simulink library "AFCToolbox"  (R2025b)
settings: Solver=VariableStepAuto  StartTime=0.0  StopTime=10.0  RelTol=1e-3
undefined symbols (not defined in the file or in its folder): AFC5Toolbox_SimuMoudle, ax, ay, az, C_d, C_dm, C_m, C_t, Control, d, declination_table, dp0, dp1, dp2, dp3, dt, euler_0, g0, I_xyz, inclination_table, J_m, lmd_high, lmd_low, lp_acc_knoise, lp_acc_max, lp_acc_min, lp_acc_seed, lp_GPS_BL_max, lp_GPS_BL_min, lp_GPS_H_max, lp_GPS_H_min, lp_GPS_knoise, lp_GPS_seed, lp_GPS_vel_max, lp_GPS_vel_min, lp_gyro_knoise, lp_gyro_max, lp_gyro_min, lp_gyro_seed, lp_hf_vwind, lp_hs_vwind_interp, lp_kaerorho, lp_kaeroT, lp_kIxyz, lp_kmass, lp_momentx_A0, lp_momentx_Af, lp_momentx_ts, lp_momenty_A0, lp_momenty_Af, lp_momenty_ts, lp_momentz_A0, lp_momentz_Af, lp_momentz_ts, lp_vf_vwind, lp_vs_vwind_interp, lp_vwind_thetax, lp_vwind_thetaz, mass, MB_states ... (+52)
libraries: $bdroot x104, simulink x75, etargetslib x32, sharedtransform x13, simulink_extras x12, dspstat3 x11, aerolibconvert2 x9, aerolibtransform2 x3, aerolibutil x2, matrix_library x1
(part 2 of 11)

== system AFCToolbox/SimuMoudle ==
  Equations of Motion1 : Subsystem  AncestorBlock=AFC5Toolbox_SimuMoudle/SimuMoudle/Equations of Motion1  mask(Equations of Motion){}
      mask init:
      | % port_label('input', 1, 'P+R+mg+F_c','texmode','on')
      | % port_label('input', 2, 'M_s_t+M_d+M_c+M\prime_r_e_l+M\prime_k','texmode','on')
      | % port_label('output', 1, 'V_G','texmode','on')
      | % port_label('output', 2, 'P_G','texmode','on')
      | % port_label('output', 3, 'R_0 _G','texmode','on')
      | % port_label('output', 4, 'G_B','texmode','on')
      | % port_label('output', 5, '\omega_T_1','texmode','on')
      | % port_label('output', 6, '\phi\prime \psi\prime \gamma\prime','texmode','on')
      | % port_label('output', 7, '\phi \psi \gamma','texmode','on')
      mask DialogControl Container1 Prompt: Equations of Motion
  Forces & Moments1 : Subsystem  AncestorBlock=AFC5Toolbox_SimuMoudle/SimuMoudle/Forces & Moments1
      mask DialogControl DescGroupVar Prompt: Forces & Moments
  LLA2XYZ : Subsystem  AncestorBlock=AFC5Toolbox_SimuMoudle/SimuMoudle/LLA2XYZ
      mask DialogControl DescGroupVar Prompt: LLA2BLH
      mask DialogControl DescTextVar Prompt: 将东北天坐标系的GPS_LLA转换为Pos_xyz
  Position-Control : Subsystem  AncestorBlock=AFC5Toolbox_SimuMoudle/SimuMoudle/Position-Control
      mask DialogControl DescGroupVar Prompt: 航线控制
      mask DialogControl DescTextVar Prompt: P0: 预设的无人机位置控制指令
  SimuBaro : Subsystem  AncestorBlock=AFC5Toolbox_SimuMoudle/SimuMoudle/SimuBaro  mask{lp_GPS_sample_time=0.01}
      mask prompts: lp_GPS_sample_time "采样时间："
      mask DialogControl DescGroupVar Prompt: 气压计模拟模块
      mask DialogControl DescTextVar Prompt: 本模块能够模拟仿真如下气压计信息：Time -- 模块时间（ms）;Press -- 气压（Pa）;H -- 高度（m）;Temp -- 温度（°）；
      mask DialogControl DescTextVar_copy Prompt: 所用时钟使用仿真时间代替；其中以下无法仿真使用常数暂代：Temp = 1;
  SimuComIn_ByteUnpack : Subsystem  AncestorBlock=AFC5Toolbox_SimuMoudle/SimuMoudle/SimuComIn_ByteUnpack  mask{para_count=4}
      mask prompts: para_count "数据位数："
      mask DialogControl DescGroupVar Prompt: SimuComIn_ByteUnpack
      mask DialogControl DescTextVar Prompt: 接收SimuCom应用层协议的数据，并分离出数据位。
  SimuComOut_BytePack : Subsystem  AncestorBlock=AFC5Toolbox_SimuMoudle/SimuMoudle/SimuComOut_BytePack
      mask DialogControl DescGroupVar Prompt: SimuComOut_BytePack
      mask DialogControl DescTextVar Prompt: 该模块将para数据位打包，适应SimuCom应用层协议。
      mask DialogControl DescTextVar_copy Prompt: para: 发送数据
  SimuGps : Subsystem  AncestorBlock=AFC5Toolbox_SimuMoudle/SimuMoudle/SimuGps  mask{lp_GPS_sample_time=0.01}
      mask prompts: lp_GPS_sample_time "采样时间："
      mask DialogControl DescGroupVar Prompt: GPS模拟模块
      mask DialogControl DescTextVar Prompt: 本模块能够模拟仿真如下GPS信息：Lat -- 维度，北纬为正（单位：°）；Lon -- 经度，东经为正（单位：°）;Alt -- 海拔高度（单位：m）;Vx -- 表示正北速度；Vy -- 表示正东速度；Vz -- 表示向上速度；Vgnd -- 地速；HeadAng -- 真北航向角（单位：°）；STS -- GPS状态；stasN -- 卫星个数；hdop -- 水平精度因子。
      mask DialogControl DescTextVar_copy Prompt: 所有时钟使用仿真时间代替；其中以下无法仿真使用常数暂代：Sts = 1;StasN = 2;hdop = 3;
  SimuICM : Subsystem  AncestorBlock=AFC5Toolbox_SimuMoudle/SimuMoudle/SimuICM  mask{lp_sample_time=0.01}
      mask prompts: lp_sample_time "采样时间："
      mask DialogControl DescGroupVar Prompt: 惯性测量模拟模块
      mask DialogControl DescTextVar Prompt: 本模块能够模拟仿真陀螺仪和加速度计如下信息：Tim -- 模拟时间（ms）；Wx Wy Wz -- 角速率（°/s）；Ax Ay Az -- 加速度（m/s^2）；Temp -- 温度（°）
      mask DialogControl Control2 Prompt: 所用时钟使用仿真时间代替；其中以下无法仿真使用常数暂代：Temp = 1;
  UAV : Subsystem  AncestorBlock=AFC5Toolbox_SimuMoudle/SimuMoudle/UAV
      mask DialogControl DescGroupVar Prompt: 无人机动力学模型
      mask DialogControl DescTextVar Prompt: 输入：w1234 -- 电机信号
      mask DialogControl DescTextVar_copy Prompt: 输出：wxyz -- 姿态角；acc -- 加速度计；BLH -- 经纬高；vel -- 速度；att -- 加速度；

== system AFCToolbox/TEST MOUDLE ==
  TEST AD/IV : Subsystem
  TEST CARD : Subsystem
  TEST LED : Subsystem
  TEST MEMS : Subsystem
  TEST POD IN : Subsystem
  TEST POD OUT : Subsystem
  TEST PORT : Subsystem
  TEST PORTDOWNLOAD : Subsystem
  TEST PWM : Subsystem
  TEST SBUS : Subsystem
  TEST SENSOR : Subsystem
  TEST SIMUCOM : Subsystem
  TEST TDEBUG : Subsystem
  TSET GPS : Subsystem

== system AFCToolbox/基础导航算法模型库 ==
  ECL EKF : Subsystem  AncestorBlock=AFC5Toolbox_SimuMoudle/TestMoudle/ECL EKF  mask{dt=0.01, inial_tim=10, static_tim=30, Parameter13=0, Parameter14=on, mag_flag=off, baro_z_flag=off, gpsvel_obsvar=[0.01,0.01,0.01], gpspos_obsvar=[0.01,0.01,0.01], obs_var_baro=0.01, R_MAG=0.25, R_decl=0.25, Parameter17=0, Parameter16=on, Parameter18=off, gpsvel_innov_gate=5, gpspos_innov_gate=5}
      mask prompts: dt "采样时间"; inial_tim "初始时间"; static_tim "静置时间"; Parameter14 "GPS使能flag"; mag_flag "磁力计使能flag"; baro_z_flag "气压计使能flag"; gpsvel_obsvar "GPSVel噪声协方差"; gpspos_obsvar "GPSPos噪声协方差"; obs_var_baro "气压计噪声协方差"; R_MAG "磁力计磁场噪声协方差"; R_decl "磁偏角噪声协方差"; Parameter16 "single"; Parameter18 "double"; gpsvel_innov_gate "位置新息一致阈值"; gpspos_innov_gate "速度新息一致阈值"
      mask DialogControl DescGroupVar Prompt: ECL EKF滤波器
      mask DialogControl DescTextVar Prompt: 基础多源信息融合导航算法模块，所融合的传感器包括陀螺仪、加速度计、多源信息 EKF 滤波、磁力计、GPS、气压计等，支持二次开发;提供专用MATLAB/Simulink工具箱并支持代码生成，用户可进行相应模块参数配置及自主建模，可参考提供的示例融合导航模型进行二次开发
      mask DialogControl Container9 Prompt: 主要
      mask DialogControl ParameterGroupVar Prompt: EKF参数
      mask DialogControl Container12 Prompt: 时间设置：
      mask DialogControl Container7 Prompt: 使能指令：
      mask DialogControl Container6 Prompt: 量测噪声协方差：
      mask DialogControl Container13 Prompt: 数据类型
      mask DialogControl Container10 Prompt: 其他

== system AFCToolbox/APPModule/AFC5StsBit ==
  AFC5Sts(UINT32) : Inport
  D0 : simulink/Logic and Bit Operations/Extract Bits  bitsToExtract=Range of bits  numBits=8  bitIdxRange=[0 0]  outScalingMode=Treat bit field as an integer
  D1 : simulink/Logic and Bit Operations/Extract Bits  bitsToExtract=Range of bits  numBits=8  bitIdxRange=[1 1]  outScalingMode=Treat bit field as an integer
  D16_D23 : simulink/Logic and Bit Operations/Extract Bits  bitsToExtract=Range of bits  numBits=8  bitIdxRange=[16 23]  outScalingMode=Treat bit field as an integer
  D2 : simulink/Logic and Bit Operations/Extract Bits  bitsToExtract=Range of bits  numBits=8  bitIdxRange=[2 2]  outScalingMode=Treat bit field as an integer
  D24_D31 : simulink/Logic and Bit Operations/Extract Bits  bitsToExtract=Range of bits  numBits=8  bitIdxRange=[24 31]  outScalingMode=Treat bit field as an integer
  D3 : simulink/Logic and Bit Operations/Extract Bits  bitsToExtract=Range of bits  numBits=8  bitIdxRange=[3 3]  outScalingMode=Treat bit field as an integer
  D4 : simulink/Logic and Bit Operations/Extract Bits  bitsToExtract=Range of bits  numBits=8  bitIdxRange=[4 4]  outScalingMode=Treat bit field as an integer
  D5 : simulink/Logic and Bit Operations/Extract Bits  bitsToExtract=Range of bits  numBits=8  bitIdxRange=[5 5]  outScalingMode=Treat bit field as an integer
  D6 : simulink/Logic and Bit Operations/Extract Bits  bitsToExtract=Range of bits  numBits=8  bitIdxRange=[6 6]  outScalingMode=Treat bit field as an integer
  D7 : simulink/Logic and Bit Operations/Extract Bits  bitsToExtract=Range of bits  numBits=8  bitIdxRange=[7 7]  outScalingMode=Treat bit field as an integer
  D8 : simulink/Logic and Bit Operations/Extract Bits  bitsToExtract=Range of bits  numBits=8  bitIdxRange=[8 8]  outScalingMode=Treat bit field as an integer
  D9_D15 : simulink/Logic and Bit Operations/Extract Bits  bitsToExtract=Range of bits  numBits=8  bitIdxRange=[9 15]  outScalingMode=Treat bit field as an integer
  Data Type Conversion{,1..8,10..11} (11 alike) : DataTypeConversion  OutDataTypeStr=boolean  SaturateOnIntegerOverflow=off  RndMeth=Floor  LockScale=on
  Data Type Conversion9 : DataTypeConversion  OutDataTypeStr=double  SaturateOnIntegerOverflow=off  RndMeth=Floor  LockScale=on
  bSystemInitSts : Outport
  bLandComplete : Outport  Port=2
  bArmedEnable : Outport  Port=3
  bDcmFast : Outport  Port=4
  bLimitRollPitch : Outport  Port=5
  bLimitYaw : Outport  Port=6
  bLimitThrottleLower : Outport  Port=7
  bLimitThrottleUpper : Outport  Port=8
  bMotorSlowStart : Outport  Port=9
  Reserved : Outport  Port=10
  iSdCardWriteErr : Outport  Port=11
  iTaskOverTimeNum : Outport  Port=12
  wires:
  D2/1 -> Data Type Conversion7/1
  D16_D23/1 -> Data Type Conversion10/1
  D1/1 -> Data Type Conversion1/1
  D0/1 -> Data Type Conversion/1
  D9_D15/1 -> Data Type Conversion9/1
  D3/1 -> Data Type Conversion6/1
  D4/1 -> Data Type Conversion5/1
  D5/1 -> Data Type Conversion4/1
  D6/1 -> Data Type Conversion3/1
  D7/1 -> Data Type Conversion2/1
  AFC5Sts(UINT32)/1 -> D0/1, D1/1, D2/1, D3/1, D4/1, D5/1, D6/1, D7/1, D8/1, D24_D31/1, D16_D23/1, D9_D15/1
  D8/1 -> Data Type Conversion8/1
  D24_D31/1 -> Data Type Conversion11/1
  Data Type Conversion/1 -> bSystemInitSts/1
  Data Type Conversion1/1 -> bLandComplete/1
  Data Type Conversion7/1 -> bArmedEnable/1
  Data Type Conversion6/1 -> bDcmFast/1
  Data Type Conversion5/1 -> bLimitRollPitch/1
  Data Type Conversion4/1 -> bLimitYaw/1
  Data Type Conversion3/1 -> bLimitThrottleLower/1
  Data Type Conversion2/1 -> bLimitThrottleUpper/1
  Data Type Conversion8/1 -> bMotorSlowStart/1
  Data Type Conversion9/1 -> Reserved/1
  Data Type Conversion10/1 -> iSdCardWriteErr/1
  Data Type Conversion11/1 -> iTaskOverTimeNum/1

== system AFCToolbox/APPModule/updateCd ==
  dcmAng : Inport
  dcmRate : Inport  Port=2
  Add : Sum
  Constant : Constant  Value=36000
  Demux : Demux  Outputs=3
  Gain : Gain  Gain=5729.5779513082320876798154814105
  Gain1 : Gain  Gain=5729.5779513082320876798154814105
  Mux : Mux  Inputs=3
  Switch : Switch  SaturateOnIntegerOverflow=off  InputSameDT=off
  attiAng : Outport
  AttiRate : Outport  Port=2
  wires:
  Gain1/1 -> AttiRate/1
  Demux/3 -> Switch/2, Switch/1, Add/1
  dcmAng/1 -> Gain/1
  Gain/1 -> Demux/1
  Add/1 -> Switch/3
  Constant/1 -> Add/2
  Switch/1 -> Mux/3
  Demux/1 -> Mux/1
  dcmRate/1 -> Gain1/1
  Mux/1 -> attiAng/1
  Demux/2 -> Mux/2

== system AFCToolbox/DeviceModule/DPS310Rst ==
  resetBarH : Inport
  DPS310 : $bdroot/DeviceModule/DPS310  Priority=1  g_sampleTime=0.01  g_comPort=6  g_instName=0  g_id=0
  DPS310Reset : S-Function  Priority=1  FunctionName=DPS310Reset  Parameters=g_sampleTime,g_comPort,g_instName,g_id  SFunctionDeploymentMode=off  EnableBusSupport=off  mask{g_sampleTime=0.01, g_comPort=6, g_instName=0, g_id=0}
      mask prompts: g_sampleTime "采样时间"
      mask DialogControl ParameterGroupVar Prompt: DPS310数字气压计模块
      mask DialogControl Control1 Prompt: 本模块能够读取数字气压计DPS310测得的压力、温度、气压高度
      mask Display: color('gray');port_label('input',1,'resetBarH');
  Tim /ms : Outport
  Press /Pa : Outport  Port=2
  Temp /°C : Outport  Port=3
  BarHeight /m : Outport  Port=4
  wires:
  resetBarH/1 -> DPS310Reset/1
  DPS310/1 -> Tim /ms/1
  DPS310/2 -> Press /Pa/1
  DPS310/3 -> Temp /°C/1
  DPS310/4 -> BarHeight /m/1

== system AFCToolbox/ServoCardModule/LED Control ==
  LED8 : Inport
  Bitwise AND : simulink/Logic and Bit Operations/Bitwise Operator  logicop=AND  UseBitMask=on  BitMask=bin2dec('00000001')  BitMaskRealWorld=Stored Integer
      settings: LibrarySourceBlock=|
      | simulink/Quick Insert/Logic and Bit
      | Operations/Bitwise AND
  Bitwise AND1 : simulink/Logic and Bit Operations/Bitwise Operator  logicop=AND  UseBitMask=on  BitMask=bin2dec('00000010')  BitMaskRealWorld=Stored Integer
      settings: LibrarySourceBlock=|
      | simulink/Quick Insert/Logic and Bit
      | Operations/Bitwise AND
  Bitwise AND2 : simulink/Logic and Bit Operations/Bitwise Operator  logicop=AND  UseBitMask=on  BitMask=4  BitMaskRealWorld=Stored Integer
      settings: LibrarySourceBlock=|
      | simulink/Quick Insert/Logic and Bit
      | Operations/Bitwise AND
  Bitwise AND3 : simulink/Logic and Bit Operations/Bitwise Operator  logicop=AND  UseBitMask=on  BitMask=8  BitMaskRealWorld=Stored Integer
      settings: LibrarySourceBlock=|
      | simulink/Quick Insert/Logic and Bit
      | Operations/Bitwise AND
  Bitwise AND4 : simulink/Logic and Bit Operations/Bitwise Operator  logicop=AND  UseBitMask=on  BitMask=16  BitMaskRealWorld=Stored Integer
      settings: LibrarySourceBlock=|
      | simulink/Quick Insert/Logic and Bit
      | Operations/Bitwise AND
  Bitwise AND5 : simulink/Logic and Bit Operations/Bitwise Operator  logicop=AND  UseBitMask=on  BitMask=32  BitMaskRealWorld=Stored Integer
      settings: LibrarySourceBlock=|
      | simulink/Quick Insert/Logic and Bit
      | Operations/Bitwise AND
  Bitwise AND6 : simulink/Logic and Bit Operations/Bitwise Operator  logicop=AND  UseBitMask=on  BitMask=64  BitMaskRealWorld=Stored Integer
      settings: LibrarySourceBlock=|
      | simulink/Quick Insert/Logic and Bit
      | Operations/Bitwise AND
  Bitwise AND7 : simulink/Logic and Bit Operations/Bitwise Operator  logicop=AND  UseBitMask=on  BitMask=128  BitMaskRealWorld=Stored Integer
      settings: LibrarySourceBlock=|
      | simulink/Quick Insert/Logic and Bit
      | Operations/Bitwise AND
  Data Type Conversion{,2..8} (8 alike) : DataTypeConversion  OutDataTypeStr=boolean  SaturateOnIntegerOverflow=off  RndMeth=Floor
  Data Type Conversion1 : DataTypeConversion  OutDataTypeStr=uint8  SaturateOnIntegerOverflow=off  RndMeth=Floor
  SeqInst : $bdroot/DeviceModule/SeqInst  Priority=6  g_chanelNo=时序指令1  g_comPort=0  g_instName=0  g_id=0
  SeqInst1 : $bdroot/DeviceModule/SeqInst  Priority=6  g_chanelNo=时序指令2  g_comPort=0  g_instName=0  g_id=0
  SeqInst2 : $bdroot/DeviceModule/SeqInst  Priority=6  g_chanelNo=时序指令3  g_comPort=0  g_instName=0  g_id=0
  SeqInst3 : $bdroot/DeviceModule/SeqInst  Priority=6  g_chanelNo=时序指令4  g_comPort=0  g_instName=0  g_id=0
  SeqInst4 : $bdroot/DeviceModule/SeqInst  Priority=6  g_chanelNo=时序指令5  g_comPort=0  g_instName=0  g_id=0
  SeqInst5 : $bdroot/DeviceModule/SeqInst  Priority=6  g_chanelNo=时序指令6  g_comPort=0  g_instName=0  g_id=0
  SeqInst6 : $bdroot/DeviceModule/SeqInst  Priority=6  g_chanelNo=时序指令7  g_comPort=0  g_instName=0  g_id=0
  SeqInst7 : $bdroot/DeviceModule/SeqInst  Priority=6  g_chanelNo=时序指令8  g_comPort=0  g_instName=0  g_id=0
  wires:
  Bitwise AND2/1 -> Data Type Conversion3/1
  LED8/1 -> Data Type Conversion1/1
  Bitwise AND5/1 -> Data Type Conversion6/1
  Bitwise AND6/1 -> Data Type Conversion7/1
  Bitwise AND1/1 -> Data Type Conversion2/1
  Bitwise AND3/1 -> Data Type Conversion4/1
  Bitwise AND7/1 -> Data Type Conversion8/1
  Bitwise AND/1 -> Data Type Conversion/1
  Bitwise AND4/1 -> Data Type Conversion5/1
  Data Type Conversion1/1 -> Bitwise AND7/1, Bitwise AND6/1, Bitwise AND5/1, Bitwise AND4/1, Bitwise AND3/1, Bitwise AND2/1, Bitwise AND1/1, Bitwise AND/1
  Data Type Conversion/1 -> SeqInst/1
  Data Type Conversion2/1 -> SeqInst1/1
  Data Type Conversion3/1 -> SeqInst2/1
  Data Type Conversion4/1 -> SeqInst3/1
  Data Type Conversion5/1 -> SeqInst4/1
  Data Type Conversion6/1 -> SeqInst5/1
  Data Type Conversion7/1 -> SeqInst6/1
  Data Type Conversion8/1 -> SeqInst7/1

== system AFCToolbox/ServoCardModule/XSimPack ==
  Parms : Inport
  Byte Pack1 : etargetslib/Byte Pack  datatypes={'uint16'}  byteAlign=1
  Byte Pack10 : etargetslib/Byte Pack  datatypes={'uint16'}  byteAlign=1
  Byte Pack6 : etargetslib/Byte Pack  datatypes={'uint32'}  byteAlign=1
  Byte Pack7 : etargetslib/Byte Pack  datatypes={'uint16'}  byteAlign=1
  Byte Pack8 : etargetslib/Byte Pack  datatypes={'single'}  byteAlign=1
  ByteCheckSum : Subsystem
  Constant1 : Constant  Value=0xDAA5
  Constant2 : Constant  Value=frameSender
  Constant3 : Constant  Value=frameType
  CounterFreeRunning2 : simulink/Sources/Counter Free-Running  NumBits=32  tsamp=-1
  Data Type Conversion1 : DataTypeConversion  OutDataTypeStr=uint16  SaturateOnIntegerOverflow=off  RndMeth=Floor
  Data Type Conversion5 : DataTypeConversion  OutDataTypeStr=uint16  SaturateOnIntegerOverflow=off  RndMeth=Floor
  Data Type Conversion6 : DataTypeConversion  OutDataTypeStr=uint32  SaturateOnIntegerOverflow=off  RndMeth=Floor
  Data Type Conversion7 : DataTypeConversion  OutDataTypeStr=uint8  SaturateOnIntegerOverflow=off  RndMeth=Floor
  Data Type Conversion8 : DataTypeConversion  OutDataTypeStr=single  SaturateOnIntegerOverflow=off  RndMeth=Floor
  Data Type Conversion9 : DataTypeConversion  OutDataTypeStr=uint16  SaturateOnIntegerOverflow=off  RndMeth=Floor
  Mux1 : Mux  Inputs=6
  Mux2 : Mux  Inputs=2
  Width2 : Width  DataType=single
  Frame : Outport
  wires:
  Data Type Conversion6/1 -> Byte Pack6/1
  Data Type Conversion9/1 -> Byte Pack10/1
  Byte Pack6/1 -> Mux1/3
  Mux1/1 -> Mux2/1, ByteCheckSum/1(In1)
  Byte Pack8/1 -> Mux1/6
  Data Type Conversion8/1 -> Byte Pack8/1
  ByteCheckSum/1(Out1) -> Mux2/2
  Byte Pack1/1 -> Mux1/2
  Data Type Conversion1/1 -> Byte Pack7/1
  Byte Pack7/1 -> Mux1/4
  Width2/1 -> Data Type Conversion5/1
  Constant2/1 -> Data Type Conversion1/1
  Byte Pack10/1 -> Mux1/1
  Data Type Conversion7/1 -> Mux1/5
  Constant1/1 -> Data Type Conversion9/1
  CounterFreeRunning2/1 -> Data Type Conversion6/1  "AseCounter"
  Constant3/1 -> Data Type Conversion7/1
  Data Type Conversion5/1 -> Byte Pack1/1
  Parms/1 -> Data Type Conversion8/1
  Mux2/1 -> Frame/1, Width2/1

== system AFCToolbox/ServoCardModule/XSimUnPack ==
  Frame : Inport
  FrameCheck : Subsystem
  Subsystem2 : Subsystem
  Terminator{1..4} (4 alike) : Terminator
  Parms : Outport
  wires:
  Subsystem2/2(SourceID) -> Terminator2/1
  Subsystem2/1(FrameCounter) -> Terminator1/1
  Subsystem2/4(FrameType) -> Terminator4/1
  Subsystem2/5(FramePara) -> Parms/1
  Subsystem2/3(TargetID) -> Terminator3/1
  Frame/1 -> FrameCheck/1(In1), Subsystem2/1(Frame)
  FrameCheck/1(Out1) -> Subsystem2/Enable

== system AFCToolbox/ServoCardModule/XSrvoCmd ==
  SrvoAng : Inport
  Mux : Mux  Inputs=2
  查询四个舵机角度指令 : Subsystem
  设置四个舵机位置与速度指令 : Subsystem
  Frame : Outport
  wires:
  Mux/1 -> Frame/1
  SrvoAng/1 -> 设置四个舵机位置与速度指令/1(Ang)
  查询四个舵机角度指令/1(RAng) -> Mux/2
  设置四个舵机位置与速度指令/1(Frame) -> Mux/1

== system AFCToolbox/ServoCardModule/XSrvoSamp ==
  note: 位置标定
  Frame : Inport
  Add{,1..3} (4 alike) : Sum
  Constant{,1..3} (4 alike) : Constant  Value=180
  Constant4 : Constant  Value=-0.0011
  Constant5 : Constant  Value=-0.0011
  Constant6 : Constant  Value=-0.0015
  Constant7 : Constant  Value=-0.0013
  Demux : Demux  Outputs=[8,8,8,8]
  Gain{,1..3} (4 alike) : Gain
  MATLAB Function : MATLAB Function  TreatAsAtomicUnit=on
  Mux : Mux
  SrvoPro : Subsystem
  SrvoPro1 : Subsystem
  SrvoPro2 : Subsystem
  SrvoPro3 : Subsystem
  Subtract{,1..3} (4 alike) : Sum  Inputs=+-
  SampAng : Outport
  wires:
  Frame/1 -> Demux/1
  Demux/4 -> SrvoPro3/1(SvoFrame)
  Demux/3 -> SrvoPro2/1(SvoFrame)
  Demux/2 -> SrvoPro1/1(SvoFrame)
  Demux/1 -> SrvoPro/1(SvoFrame)
  Mux/1 -> SampAng/1
  Subtract/1 -> Gain/1
  Constant/1 -> Subtract/2
  Constant1/1 -> Subtract1/2
  MATLAB Function/2(out2) -> Subtract1/1
  Constant2/1 -> Subtract2/2
  MATLAB Function/3(out3) -> Subtract2/1
  Constant3/1 -> Subtract3/2
  MATLAB Function/4(out4) -> Subtract3/1
  Constant4/1 -> Add/2
  Gain/1 -> Add/1
  Add/1 -> Mux/1
  Gain1/1 -> Add1/1
  Constant5/1 -> Add1/2
  Subtract1/1 -> Gain1/1
  Subtract2/1 -> Gain2/1
  Constant6/1 -> Add2/2
  Gain2/1 -> Add2/1
  Gain3/1 -> Add3/1
  Constant7/1 -> Add3/2
  Subtract3/1 -> Gain3/1
  Add1/1 -> Mux/2
  Add2/1 -> Mux/3
  Add3/1 -> Mux/4
  SrvoPro/1(ID) -> MATLAB Function/1(ID1)
  SrvoPro/2(angleACK) -> MATLAB Function/2(angleACK1)
  MATLAB Function/1(out1) -> Subtract/1
  SrvoPro1/1(ID) -> MATLAB Function/3(ID2)
  SrvoPro1/2(angleACK) -> MATLAB Function/4(angleACK2)
  SrvoPro2/1(ID) -> MATLAB Function/5(ID3)
  SrvoPro2/2(angleACK) -> MATLAB Function/6(angleACK3)
  SrvoPro3/1(ID) -> MATLAB Function/7(ID4)
  SrvoPro3/2(angleACK) -> MATLAB Function/8(angleACK4)

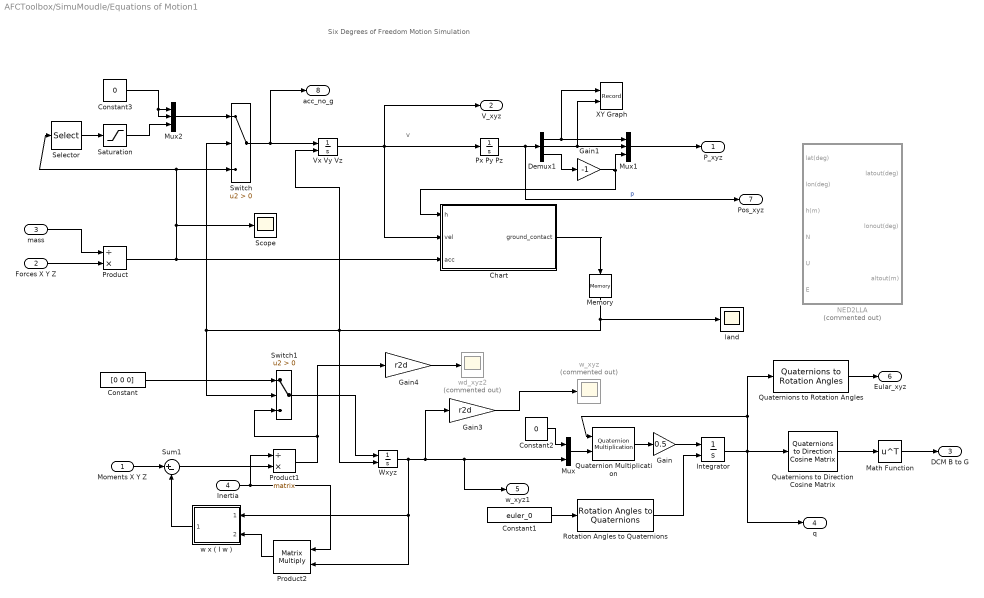
== system AFCToolbox/SimuMoudle/Equations of Motion1 ==
  note: Six Degrees of Freedom Motion Simulation
  note: v
  Moments X Y Z : Inport
  Forces X Y Z : Inport  Port=2
  mass : Inport  Port=3
  Inertia : Inport  Port=4
  Chart : Stateflow chart  TreatAsAtomicUnit=on
  Constant : Constant  Value=[0 0 0]
  Constant1 : Constant  Value=euler_0
  Constant2 : Constant  Value=0
  Constant3 : Constant  Value=0
  Demux1 : Demux  Outputs=3
  Gain : Gain  Gain=0.5
  Gain1 : Gain  Gain=-1
  Gain3 : Gain  Gain=r2d
  Gain4 : Gain  Gain=r2d
  Integrator : Integrator  InitialConditionSource=external  InitialCondition=[1 0 0 0]
  Math Function : Math  Operator=transpose  SignedPower=on
  Memory : Memory
  Mux : Mux  Inputs=2
  Mux1 : Mux  Inputs=3
  Mux2 : Mux  Inputs=3
  NED2LLA : Subsystem  Commented=on
  Product : Product  Inputs=/*  RndMeth=Zero
  Product1 : Product  Inputs=/*  Multiplication=Matrix(*)  RndMeth=Zero
  Product2 : Product  Multiplication=Matrix(*)  RndMeth=Zero
  Px Py Pz : Integrator  InitialCondition=[0,0,0]
  Quaternion Multiplication : aerolibutil/Quaternion Multiplication
  Quaternions to Direction Cosine Matrix : sharedtransform/Quaternions to  Direction Cosine Matrix  aMode=aMode
  Quaternions to Rotation Angles : sharedtransform/Quaternions to Rotation Angles  rotationOrder=ZYX  aMode=aMode
  Rotation Angles to Quaternions : sharedtransform/Rotation Angles to Quaternions  rotationOrder=ZYX  aMode=aMode
  Saturation : Saturate  UpperLimit=0  LowerLimit=-inf
  Scope : Scope
      settings: ActiveDisplayYMinimum=-26.03097  ActiveDisplayYMaximum=21.745
  Selector : Selector  InputPortWidth=3  IndexOptions=Index vector (dialog)  Indices=[3]  OutputSizes=1
  Sum1 : Sum  Inputs=|+-
  Switch : Switch  Criteria=u2 > Threshold  SaturateOnIntegerOverflow=off  InputSameDT=off
  Switch1 : Switch  Criteria=u2 > Threshold  SaturateOnIntegerOverflow=off  InputSameDT=off
  Vx Vy Vz : Integrator  ExternalReset=level  InitialCondition=velocity_0
  Wxyz : Integrator  ExternalReset=level  InitialCondition=omega_0
  XY Graph : Record  NumPorts=2.0  FileSettingsInternal="{\"entries\":[{\"content\":{\"excelSettings\":{\"content\":{},\"type\":\"Streamout.ExcelSettings\"},\"parquetSettings\":{\"content\":{},\"type\":\"Streamout.ParquetSettings\"}},\"type\":\"Streamout.FileSettingStorage\",\"uuid\":\"\"}],\"packageUris\":[\"http:\\/\\/schema.mathworks.com\\/mf0\\/streamout_blocks\\/R2020a\"],\"version\":\"1.0\"}"  FrameSettings=[0, 0]  Layout=[1 1]  SignalsInternal="{\"entries\":[{\"content\":{},\"type\":\"RecordBlkView.InputSignals\",\"uuid\":\"\"}],\"packageUris\":[\"http:\\/\\/schema.mathworks.com\\/mf0\\/streamout_blocks\\/R2020a\"],\"version\":\"1.0\"}"  VisualizationBindings="{\"sparklinesplugin\":{\"info\":[{\"bindingParametersList\":[],\"subplotID\":1}]}}"  CompatibilityTag=XY  st=-1
  land : Scope
      settings: ActiveDisplayYMinimum=-0.125  ActiveDisplayYMaximum=1.125  DataLoggingVariableName=ScopeData7
  w x ( I w ) : Subsystem  mask(Cross Product){}
      mask help: [a;b;c] x [x;y;z] = [bz-cy; cx-az; ay-bx]
      mask Display: fprintf('Cross\nProduct')
  w_xyz : Scope  Commented=on
      settings: TimeSpan=30  ActiveDisplayYMinimum=-154.64672  ActiveDisplayYMaximum=154.53713  DataLoggingVariableName=SD_w  DataLoggingSaveFormat=Array
  wd_xyz2 : Scope  Commented=on
      settings: TimeSpan=30  ActiveDisplayYMinimum=-10265.36258  ActiveDisplayYMaximum=10256.64919  DataLoggingVariableName=Position_Scope13  DataLoggingSaveFormat=Array
  P_xyz : Outport  InitialOutput=0
  V_xyz : Outport  Port=2  InitialOutput=0
  DCM B to G : Outport  Port=3  InitialOutput=0
  q : Outport  Port=4  InitialOutput=0
  w_xyz1 : Outport  Port=5  InitialOutput=0
  Eular_xyz : Outport  Port=6  InitialOutput=0
  Pos_xyz : Outport  Port=7  InitialOutput=0
  acc_no_g : Outport  Port=8  InitialOutput=0
  wires:
  Product2/1 -> w x ( I w )/2(b(1) b(2) b(3))
  Inertia/1 -> Product2/1, Product1/1
  Sum1/1 -> Product1/2
  Forces X Y Z/1 -> Product/2
  mass/1 -> Product/1
  Product1/1 -> Gain4/1, Switch1/3
  Quaternions to Direction Cosine Matrix/1 -> Math Function/1
  Gain3/1 -> w_xyz/1
  Gain4/1 -> wd_xyz2/1
  w x ( I w )/1(c(1) c(2) c(3)) -> Sum1/2
  Vx Vy Vz/1 -> Chart/2(vel), Px Py Pz/1, V_xyz/1
  Wxyz/1 -> w x ( I w )/1(a(1) a(2) a(3)), Product2/2, Gain3/1, w_xyz1/1, Mux/2
  Moments X Y Z/1 -> Sum1/1
  Constant2/1 -> Mux/1
  Mux/1 -> Quaternion Multiplication/2
  Quaternion Multiplication/1 -> Gain/1
  Gain/1 -> Integrator/1
  Rotation Angles to Quaternions/1 -> Integrator/2
  Constant1/1 -> Rotation Angles to Quaternions/1
  Quaternions to Rotation Angles/1 -> Eular_xyz/1
  Demux1/1 -> XY Graph/1, Mux1/1
  Demux1/2 -> XY Graph/2, Mux1/2
  Gain1/1 -> Mux1/3, Chart/1(h)
  Demux1/3 -> Gain1/1
  Px Py Pz/1 -> Pos_xyz/1, Demux1/1  "p"
  Product/1 -> Scope/1, Selector/1, Switch/3, Chart/3(acc)
  Chart/1(ground_contact) -> Memory/1
  Memory/1 -> Wxyz/2, Switch1/2, Switch/2, Vx Vy Vz/2, land/1
  Constant3/1 -> Mux2/2, Mux2/1
  Selector/1 -> Saturation/1
  Saturation/1 -> Mux2/3
  Mux2/1 -> Switch/1
  Switch/1 -> acc_no_g/1, Vx Vy Vz/1
  Constant/1 -> Switch1/1
  Math Function/1 -> DCM B to G/1
  Integrator/1 -> Quaternions to Direction Cosine Matrix/1, Quaternion Multiplication/1, Quaternions to Rotation Angles/1, q/1
  Switch1/1 -> Wxyz/1
  Mux1/1 -> P_xyz/1

== system AFCToolbox/SimuMoudle/Forces & Moments1 ==
  acc_no_g : Inport
  B to G : Inport  Port=2
  V_xyz : Inport  Port=3
  w1234 : Inport  Port=4
  xyz : Inport  Port=5
  w_xyz1 : Inport  Port=6
  Forces : Subsystem
  Moments : Subsystem
  Parameters : Subsystem
      mask init:
      | % port_label('input', 1, '\delta_x_ _c \delta_y_ _c \delta_z_ _c','texmode','on')
      | % port_label('output', 1, '\delta_x \delta_y \delta_z','texmode','on')
  acc_body : Subsystem
  F : Outport
  M : Outport  Port=2
  mass : Outport  Port=3
  Inertia : Outport  Port=4
  acc : Outport  Port=5
  wires:
  Forces/1("F ") -> F/1
  Moments/1(M) -> M/1
  xyz/1 -> Parameters/2(xyz)
  V_xyz/1 -> Parameters/1(V_xyz)
  w_xyz1/1 -> Moments/1(w_xyz1)
  Parameters/2(mass) -> mass/1, Forces/4(mass)
  Parameters/1(Vb_a) -> Forces/3(Vb_a)
  w1234/1 -> Moments/2(w_1234), Forces/2(w1234)
  B to G/1 -> acc_body/1(B2G), Forces/1(B to G), Parameters/3(B to G)
  Parameters/4(g) -> acc_body/2(g), Forces/5(g)
  Parameters/3(Inertia) -> Inertia/1
  acc_no_g/1 -> acc_body/3(acc_no_g)
  acc_body/1(acc) -> acc/1

== system AFCToolbox/SimuMoudle/LLA2XYZ ==
  gpspos_ori : Inport
  Angle Conversion1 : aerolibconvert2/Angle Conversion  IU=rad  OU=deg
  Angle Conversion2 : aerolibconvert2/Angle Conversion  IU=rad  OU=deg
  Bus Creator2 : BusCreator  Inputs=3
  LLA2NED : Subsystem
  command word10 : Constant  Value=0.402497166193948
  command word11 : Constant  Value=500
  command word9 : Constant  Value=1.978927027963337
  "sensorout " : Outport
  wires:
  command word10/1 -> Angle Conversion1/1  "lat"
  gpspos_ori/1 -> LLA2NED/2(LLA)
  Bus Creator2/1 -> LLA2NED/1(LLA0)
  LLA2NED/1("sensorout ") -> "sensorout "/1
  command word11/1 -> Bus Creator2/3  "alt"
  Angle Conversion2/1 -> Bus Creator2/1  "lon"
  Angle Conversion1/1 -> Bus Creator2/2  "lat"
  command word9/1 -> Angle Conversion2/1  "lon"

== system AFCToolbox/SimuMoudle/Position-Control ==
  Enable : EnablePort
  "Consistent formation control " : Subsystem
  From : From  Commented=on  GotoTag=p0_k
  From12 : From  Commented=on  GotoTag=v1_k
  From13 : From  Commented=on  GotoTag=v2_k
  From14 : From  Commented=on  GotoTag=v3_k
  From15 : From  Commented=on  GotoTag=w0_k
  From16 : From  Commented=on  GotoTag=w1_k
  From17 : From  Commented=on  GotoTag=w2_k
  From18 : From  Commented=on  GotoTag=w3_k
  From19 : From  Commented=on  GotoTag=W0_k
  From20 : From  Commented=on  GotoTag=W1_k
  From21 : From  Commented=on  GotoTag=W2_k
  From22 : From  Commented=on  GotoTag=W3_k
  From4 : From  Commented=on  GotoTag=p1_k
  From5 : From  Commented=on  GotoTag=p2_k
  From6 : From  Commented=on  GotoTag=p3_k
  From8 : From  Commented=on  GotoTag=v0_k
  Leader : Subsystem
  Mux{,1..3} (4 alike) : Mux  Commented=on
  Scope{,1..3} (4 alike) : Scope  Commented=on
      Scope settings: ActiveDisplayYMinimum=-682.9421  ActiveDisplayYMaximum=445.48974  DataLoggingVariableName=P  DataLoggingSaveFormat=Structure
      Scope1 settings: ActiveDisplayYMinimum=1.84996  ActiveDisplayYMaximum=4.82857  DataLoggingVariableName=V  DataLoggingSaveFormat=Structure
      Scope2 settings: ActiveDisplayYMinimum=-5.09733  ActiveDisplayYMaximum=3.44424  DataLoggingVariableName=w  DataLoggingSaveFormat=Structure
      Scope3 settings: ActiveDisplayYMinimum=-2.51477  ActiveDisplayYMaximum=3.67983  DataLoggingVariableName=W  DataLoggingSaveFormat=Structure
  P0 : Outport
  tag scope: W0_k=global, X0_k_1=global, p0_k=global, u=global, v0_k=global, w0_k=global
  wires:
  Leader/6(W0_k) -> [W0_k]
  "Consistent formation control "/1(u) -> [u]
  Leader/3(X0_k_1) -> [X0_k_1]
  [u0_k] -> "Consistent formation control "/1(u0_k)
  [X2_k_1] -> "Consistent formation control "/3(X2_k_1)
  [X0_k_1] -> "Consistent formation control "/5(X0_k_1)
  [X3_k_1] -> "Consistent formation control "/4(X3_k_1)
  Leader/1(p0_k) -> [p0_k], P0/1
  From19/1 -> Mux3/1
  Mux3/1 -> Scope3/1
  Leader/2(u0_k——xyz加速度) -> [u0_k]
  From15/1 -> Mux2/1
  From13/1 -> Mux1/3
  From8/1 -> Mux1/1
  From16/1 -> Mux2/2
  From22/1 -> Mux3/4
  From14/1 -> Mux1/4
  From21/1 -> Mux3/3
  From12/1 -> Mux1/2
  [X1_k_1] -> "Consistent formation control "/2(X1_k_1)
  Mux/1 -> Scope/1
  From20/1 -> Mux3/2
  From4/1 -> Mux/2  "p1"
  From5/1 -> Mux/3  "p2"
  Leader/4(v0_k) -> [v0_k]
  Mux1/1 -> Scope1/1
  From17/1 -> Mux2/3
  From6/1 -> Mux/4  "p3"
  Mux2/1 -> Scope2/1
  From/1 -> Mux/1  "p0"
  From18/1 -> Mux2/4
  Leader/5(w0_k) -> [w0_k]

== system AFCToolbox/SimuMoudle/SimuBaro ==
  Pos_xyz : Inport
  Baro model : Subsystem
  Digital Clock : DigitalClock
  Selector : Selector  InputPortWidth=3  IndexOptions=Index vector (dialog)  Indices=[3]  OutputSizes=1
  Tim/ms : Outport
  Press/Pa : Outport  Port=2
  "H " : Outport  Port=3
  Temp/° : Outport  Port=4
  wires:
  Selector/1 -> "H "/1
  Digital Clock/1 -> Tim/ms/1
  Baro model/1(Pa out) -> Press/Pa/1
  Baro model/2(Tem out) -> Temp/°/1
  Pos_xyz/1 -> Baro model/1(H), Selector/1

== system AFCToolbox/SimuMoudle/SimuComIn_ByteUnpack ==
  In : Inport
  Byte Unpack1 : etargetslib/Byte Unpack  dimensions={1,1,1,1,1,1,[para_count],1}  datatypes={'uint16','uint16','uint32','uint8','uint8','uint8','single','uint8'}  byteAlign=1
  Terminator{,2..7} (7 alike) : Terminator
  para : Outport
  wires:
  Byte Unpack1/7 -> para/1
  In/1 -> Byte Unpack1/1
  Byte Unpack1/6 -> Terminator6/1
  Byte Unpack1/8 -> Terminator7/1
  Byte Unpack1/4 -> Terminator4/1
  Byte Unpack1/3 -> Terminator3/1
  Byte Unpack1/2 -> Terminator2/1
  Byte Unpack1/5 -> Terminator5/1
  Byte Unpack1/1 -> Terminator/1

== system AFCToolbox/SimuMoudle/SimuComOut_BytePack ==
  para : Inport
  Byte Pack1 : etargetslib/Byte Pack  datatypes={'uint16','uint16','uint32','uint8','uint8','uint8','single'}  byteAlign=1
  CheckSum : Subsystem
  Constant1 : Constant  Value=hex2dec('DAA5')  SampleTime=-1
  Constant6 : Constant  Value=hex2dec('1')  SampleTime=-1
  Constant7 : Constant  Value=hex2dec('22')  SampleTime=-1
  Constant8 : Constant  Value=hex2dec('50')  SampleTime=-1
  Counter Free-Running1 : simulink/Sources/Counter Free-Running  NumBits=32  tsamp=-1
  Data Type Conversion1 : DataTypeConversion  OutDataTypeStr=single  SaturateOnIntegerOverflow=off  RndMeth=Floor
  Data Type Conversion4 : DataTypeConversion  OutDataTypeStr=uint16  SaturateOnIntegerOverflow=off  RndMeth=Floor
  Data Type Conversion5 : DataTypeConversion  OutDataTypeStr=uint32  SaturateOnIntegerOverflow=off  RndMeth=Floor
  Data Type Conversion6 : DataTypeConversion  OutDataTypeStr=uint16  SaturateOnIntegerOverflow=off  RndMeth=Floor
  Data Type Conversion7 : DataTypeConversion  OutDataTypeStr=uint8  SaturateOnIntegerOverflow=off  RndMeth=Floor
  Data Type Conversion8 : DataTypeConversion  OutDataTypeStr=uint8  SaturateOnIntegerOverflow=off  RndMeth=Floor
  Data Type Conversion9 : DataTypeConversion  OutDataTypeStr=uint8  SaturateOnIntegerOverflow=off  RndMeth=Floor
  Mux1 : Mux  Inputs=2
  Width : Width
  Out : Outport
  wires:
  Data Type Conversion1/1 -> Byte Pack1/7
  Width/1 -> Data Type Conversion4/1
  Data Type Conversion9/1 -> Byte Pack1/6  "frameType"
  Byte Pack1/1 -> CheckSum/1(In1), Mux1/1
  Data Type Conversion8/1 -> Byte Pack1/5  "sendIDT"
  Constant6/1 -> Data Type Conversion7/1
  Constant8/1 -> Data Type Conversion9/1
  Data Type Conversion4/1 -> Byte Pack1/2  "frameLengthT"
  Constant1/1 -> Data Type Conversion6/1
  Data Type Conversion5/1 -> Byte Pack1/3  "frameTimeT"
  Constant7/1 -> Data Type Conversion8/1
  Data Type Conversion6/1 -> Byte Pack1/1  "frameHeadT"
  Data Type Conversion7/1 -> Byte Pack1/4  "sendIDT"
  Counter Free-Running1/1 -> Data Type Conversion5/1
  CheckSum/1(Out1) -> Mux1/2
  para/1 -> Data Type Conversion1/1
  Mux1/1 -> Width/1, Out/1

== system AFCToolbox/SimuMoudle/SimuGps ==
  Pos_xyz : Inport
  Vel : Inport  Port=2
  Constant : Constant
  Constant1 : Constant  Value=2
  Constant2 : Constant  Value=3
  Demux : Demux  Outputs=3
  Demux1 : Demux  Outputs=3
  Digital Clock : DigitalClock
  Digital Clock1 : DigitalClock
  LLA model : Subsystem
  Rate Transition : RateTransition  OutPortSampleTime=lp_GPS_sample_time
  Rate Transition1 : RateTransition  OutPortSampleTime=lp_GPS_sample_time
  Vel model : Subsystem
  GPSTim/s : Outport
  lat/° : Outport  Port=2
  lon/° : Outport  Port=3
  Alt/m : Outport  Port=4
  Vx/m/s : Outport  Port=5
  Vy/m/s : Outport  Port=6
  Vz/m/s : Outport  Port=7
  Vgnd/m/s : Outport  Port=8
  Head/° : Outport  Port=9
  Sts : Outport  Port=10
  StasN : Outport  Port=11
  hdop : Outport  Port=12
  AFCTim/ms : Outport  Port=13
  wires:
  Digital Clock1/1 -> AFCTim/ms/1
  Constant2/1 -> hdop/1
  Constant1/1 -> StasN/1
  Constant/1 -> Sts/1
  Demux1/3 -> Vz/m/s/1
  Demux1/2 -> Vy/m/s/1
  Demux1/1 -> Vx/m/s/1
  Digital Clock/1 -> GPSTim/s/1
  Vel model/3(Psi_GPS_航向角) -> Head/°/1
  Demux/2 -> lon/°/1  "lon"
  Demux/1 -> lat/°/1  "lat"
  Pos_xyz/1 -> Rate Transition/1
  LLA model/1(LLA out) -> Demux/1
  Rate Transition/1 -> LLA model/1(xyz)
  Vel/1 -> Rate Transition1/1
  Rate Transition1/1 -> Vel model/1(Vel_GPS)
  Vel model/2(Vg_地速) -> Vgnd/m/s/1
  Demux/3 -> Alt/m/1  "Alt"
  Vel model/1(Vel_GPS out) -> Demux1/1

== system AFCToolbox/SimuMoudle/SimuICM ==
  wxyz : Inport
  acc : Inport  Port=2
  Constant : Constant
  Demux : Demux  Outputs=3
  Demux1 : Demux  Outputs=3
  Digital Clock : DigitalClock
  acclerate  model2 : Subsystem
  gyro model1 : Subsystem
  Tim/ms : Outport
  Wx/°/s : Outport  Port=2
  Wy/°/s : Outport  Port=3
  Wz/°/s : Outport  Port=4
  Ax/m/s^2 : Outport  Port=5
  Ay/m/s^2 : Outport  Port=6
  Az/m/s^2 : Outport  Port=7
  Temp/° : Outport  Port=8
  wires:
  Digital Clock/1 -> Tim/ms/1
  Constant/1 -> Temp/°/1
  Demux/3 -> Wz/°/s/1
  Demux/2 -> Wy/°/s/1
  Demux1/3 -> Az/m/s^2/1
  Demux1/2 -> Ay/m/s^2/1
  acc/1 -> acclerate  model2/1(axyz)
  wxyz/1 -> gyro model1/1(wxyz)
  Demux1/1 -> Ax/m/s^2/1
  gyro model1/1(gyro out) -> Demux/1
  acclerate  model2/1(accel out) -> Demux1/1
  Demux/1 -> Wx/°/s/1

== system AFCToolbox/SimuMoudle/UAV ==
  note: Six Degree of Freedom for GNC System Simulation
  note: 需求：
      | 1.无人机的轨迹过程含有GPS和拒止两个环境。
      | 2.无人机相对信息模拟，括相对距离和方向+噪声；
      | 3.拒止环境下，利用相对距离和方向信息建立的协同定位模型，解算各个无人机位置，再替代GPS信息进行无人机修正；
  w1234 : Inport
  Equations of Motion : Subsystem  mask(Equations of Motion){}
      mask init: same as AFCToolbox/SimuMoudle/Equations of Motion1
  Forces & Moments : Subsystem
  Gain1 : Gain  Gain=r2d
  Scope : Scope
      settings: ActiveDisplayYMinimum=-380.38187  ActiveDisplayYMaximum=3423.43216  DataLoggingVariableName=ScopeData2
  Scope1 : Scope
      settings: ActiveDisplayYMinimum=-29.07567  ActiveDisplayYMaximum=3.23063  DataLoggingVariableName=ScopeData3
  Scope2 : Scope
      settings: ActiveDisplayYMinimum=-3423.43216  ActiveDisplayYMaximum=380.38187
  Subsystem3 : Subsystem
  Terminator1 : Terminator
  wxyz : Outport
  acc : Outport  Port=2
  Pos_xyz : Outport  Port=3
  Vel : Outport  Port=4
  att : Outport  Port=5
  wires:
  Equations of Motion/2(V_xyz) -> Vel/1, Forces & Moments/3(V_xyz), Scope1/1
  Equations of Motion/6(Eular_xyz) -> Gain1/1
  Gain1/1 -> att/1
  Subsystem3/1(Out1) -> Scope2/1
  Forces & Moments/1(F) -> Equations of Motion/2(Forces X Y Z)
  Forces & Moments/2(M) -> Equations of Motion/1(Moments X Y Z)
  Equations of Motion/3(DCM B to G) -> Forces & Moments/2(B to G)
  w1234/1 -> Forces & Moments/4(w1234)
  Forces & Moments/3(mass) -> Equations of Motion/3(mass)
  Forces & Moments/4(Inertia) -> Equations of Motion/4(Inertia)
  Equations of Motion/4(q) -> Terminator1/1
  Equations of Motion/8(acc_no_g) -> Forces & Moments/1(acc_no_g)
  Equations of Motion/5(w_xyz1) -> wxyz/1, Forces & Moments/6(w_xyz1)
  Forces & Moments/5(acc) -> acc/1
  Equations of Motion/7(BLH) -> Pos_xyz/1
  Equations of Motion/1(P_xyz) -> Scope/1, Subsystem3/1(Pos), Forces & Moments/5(xyz)

== system AFCToolbox/TEST MOUDLE/TEST AD//IV ==
  AdSample : $bdroot/DeviceModule/AdSample  Priority=1  g_sampleTime=0.01  g_comPort=0  g_instName=0  g_id=0
  Add : Sum  Inputs=+-
  Constant12 : Constant  Value=-6.34
  Constant14 : Constant  Value=352
  Constant15 : Constant  Value=13.43
  DTComOut : $bdroot/DeviceModule/DTComOut  Priority=8  g_frameType=1  g_outFreq=1  g_comPort=0  g_instName=0  g_id=0
  Divide : Product  Inputs=*/
  Gain : Gain  Gain=100
  HiEscCmd5 : $bdroot/DeviceModule/HiEscCmd  Priority=6  g_chanelNo=1  g_minPW=40  g_maxPW=80  g_comPort=6  g_instName=0  g_id=0
  HiEscCmd6 : $bdroot/DeviceModule/HiEscCmd  Priority=6  g_chanelNo=9  g_minPW=40  g_maxPW=80  g_comPort=6  g_instName=0  g_id=0
  HiEscCmd7 : $bdroot/DeviceModule/HiEscCmd  Priority=6  g_chanelNo=7  g_minPW=40  g_maxPW=80  g_comPort=6  g_instName=0  g_id=0
  HiEscCmd8 : $bdroot/DeviceModule/HiEscCmd  Priority=6  g_chanelNo=2  g_minPW=40  g_maxPW=80  g_comPort=6  g_instName=0  g_id=0
  Moving Average : dspstat3/Moving Average  Method=Exponential weighting  ForgettingFactorPort=off  SpecifyWindowLength=on  WindowLength=4  OverlapLength=3  AllowArbitraryInputLength=off  ForgettingFactor=0.8  SimulateUsing=Code generation
  Moving Average1 : dspstat3/Moving Average  Method=Exponential weighting  ForgettingFactorPort=off  SpecifyWindowLength=on  WindowLength=4  OverlapLength=3  AllowArbitraryInputLength=off  ForgettingFactor=0.8  SimulateUsing=Code generation
  NOT : Logic  Operator=NOT  IconShape=distinctive  AllPortsSameDT=off  OutDataTypeStr=boolean
  Product : Product
  SBusCmd3 : $bdroot/DeviceModule/SBusCmd  Priority=0  g_sampleTime=T_c  g_chanelNo=3  g_comPort=6  g_instName=0  g_id=0
  Subsystem3 : Subsystem
  Sum : Sum  Inputs=|++
  Terminator : Terminator
  tag scope: pwm=global
  wires:
  NOT/1 -> Subsystem3/Enable
  Constant14/1 -> Add/2
  Sum/1 -> Moving Average/1  "I/A(y)"
  Divide/1 -> HiEscCmd5/1, HiEscCmd6/1, HiEscCmd7/1, HiEscCmd8/1, [pwm]
  AdSample/3 -> Moving Average1/1  "V/v"
  Gain/1 -> Subsystem3/1(Input), Product/2
  Add/1 -> Divide/1
  Moving Average1/1 -> Terminator/1
  [pwm] -> NOT/1
  Moving Average/1 -> DTComOut/1  "I/A"
  Constant12/1 -> Product/1
  Product/1 -> Sum/2
  AdSample/2 -> Gain/1  "I/A"
  Constant15/1 -> Divide/2
  SBusCmd3/1 -> Add/1
  [b] -> Sum/1
  Subsystem3/1(1) -> [b]

== system AFCToolbox/TEST MOUDLE/TEST CARD ==
  AFCTimer : $bdroot/DeviceModule/AFCTimer  Priority=0  g_sampleTime=0.01  g_comPort=6  g_instName=0  g_id=0
  ICM42688 : $bdroot/DeviceModule/ICM42688  Priority=0  g_sampleTime=0.01  g_comPort=6  g_instName=0  g_id=0
  Mux : Mux  Inputs=5
  SDCard1 : $bdroot/DeviceModule/SDCard  Priority=8  g_taskName=F  g_varName=time,ax,ay,az,temp  g_outFreq=5  g_comPort=0  g_instName=0  g_id=0
  wires:
  ICM42688/8 -> Mux/5
  Mux/1 -> SDCard1/1
  AFCTimer/1 -> Mux/1
  ICM42688/5 -> Mux/2
  ICM42688/7 -> Mux/4
  ICM42688/6 -> Mux/3

== system AFCToolbox/TEST MOUDLE/TEST LED ==
  Data Type Conversion5 : DataTypeConversion  OutDataTypeStr=boolean  SaturateOnIntegerOverflow=off  RndMeth=Floor
  LedGroup : $bdroot/DeviceModule/LedGroup  Priority=7  g_frameType=0  g_comPort=6  g_instName=0  g_id=0
  Pulse Generator1 : DiscretePulseGenerator  PulseType=Time based  Period=1  PulseWidth=50
  wires:
  Data Type Conversion5/1 -> LedGroup/2, LedGroup/4, LedGroup/3, LedGroup/1
  Pulse Generator1/1 -> Data Type Conversion5/1

== system AFCToolbox/TEST MOUDLE/TEST MEMS ==
  note: ICM42688
  note: ICM20602
  DTComOut1 : $bdroot/DeviceModule/DTComOut  Priority=8  g_frameType=3  g_outFreq=10  g_comPort=0  g_instName=0  g_id=0
  ICM20602 : $bdroot/DeviceModule/ICM20602  Priority=0  g_sampleTime=0.002  g_comPort=6  g_instName=0  g_id=0
  ICM42688 : $bdroot/DeviceModule/ICM42688  Priority=0  g_sampleTime=0.002  g_comPort=6  g_instName=0  g_id=0
  Mux3 : Mux  Inputs=16
  wires:
  ICM20602/4 -> Mux3/4  "ICM2_Wz"
  Mux3/1 -> DTComOut1/1
  ICM20602/6 -> Mux3/6  "ICM2_Ay"
  ICM42688/7 -> Mux3/15  "ICM4_Az"
  ICM42688/3 -> Mux3/11  "ICM4_Wy"
  ICM20602/3 -> Mux3/3  "ICM2_Wy"
  ICM20602/1 -> Mux3/1  "ICM2_Tim"
  ICM20602/2 -> Mux3/2  "ICM2_Wx"
  ICM20602/8 -> Mux3/8  "ICM2_Temp"
  ICM20602/7 -> Mux3/7  "ICM2_Az"
  ICM42688/1 -> Mux3/9  "ICM_Tim"
  ICM42688/4 -> Mux3/12  "ICM4_Wz"
  ICM42688/2 -> Mux3/10  "ICM4_Wx"
  ICM20602/5 -> Mux3/5  "ICM2_Ax"
  ICM42688/5 -> Mux3/13  "ICM4_Ax"
  ICM42688/6 -> Mux3/14  "ICM4_Ay"
  ICM42688/8 -> Mux3/16  "ICM4_Temp"

== system AFCToolbox/TEST MOUDLE/TEST POD IN ==
  BytePack1 : etargetslib/Byte Pack  datatypes={'uint8','uint8','uint8','int16','int16','uint8','int8','int8','int8','int8','int8','int8','int8'}  byteAlign=1
  ComXOut1 : $bdroot/DeviceModule/ComXOut  Priority=8  g_comPort=UART7(RS232)  g_baudRate=115200  g_outFreq=1
  Constant10 : Constant  Value=-50  SampleTime=-1
  Constant11 : Constant  Value=hex2dec('00')  SampleTime=-1
  Constant12 : Constant  Value=hex2dec('00')  SampleTime=-1
  Constant13 : Constant  Value=hex2dec('00')  SampleTime=-1
  Constant5 : Constant  Value=hex2dec('EB')  SampleTime=-1
  Constant7 : Constant  Value=hex2dec('90')  SampleTime=-1
  Constant9 : Constant  Value=hex2dec('3B')  SampleTime=-1
  DTComOut1 : $bdroot/DeviceModule/DTComOut  Priority=8  g_frameType=2  g_outFreq=1  g_comPort=0  g_instName=0  g_id=0
  Data Type Conversion{1,3,14..15} (4 alike) : DataTypeConversion  OutDataTypeStr=uint8  SaturateOnIntegerOverflow=off  RndMeth=Floor
  Data Type Conversion12 : DataTypeConversion  OutDataTypeStr=int16  SaturateOnIntegerOverflow=off  RndMeth=Floor
  Data Type Conversion13 : DataTypeConversion  OutDataTypeStr=int16  SaturateOnIntegerOverflow=off  RndMeth=Floor
  Data Type Conversion16 : DataTypeConversion  OutDataTypeStr=int8  SaturateOnIntegerOverflow=off  RndMeth=Floor
  Data Type Conversion2 : DataTypeConversion  OutDataTypeStr=int8  SaturateOnIntegerOverflow=off  RndMeth=Floor
  Gain2 : Gain  Gain=100
  Gain3 : Gain  Gain=100
  Mux2 : Mux  Inputs=2
  Sine Wave1 : Sin  SineType=Sample based  Amplitude=100  Samples=10000  SampleTime=0.01
  Subsystem1 : Subsystem
  wires:
  Data Type Conversion16/1 -> BytePack1/8, BytePack1/9, BytePack1/10, BytePack1/11, BytePack1/13, BytePack1/12
  Mux2/1 -> ComXOut1/1
  Gain2/1 -> Data Type Conversion12/1
  Constant7/1 -> Data Type Conversion15/1
  Constant9/1 -> Data Type Conversion3/1
  Data Type Conversion15/1 -> BytePack1/2
  Data Type Conversion14/1 -> BytePack1/6
  Data Type Conversion3/1 -> BytePack1/3
  Sine Wave1/1 -> DTComOut1/1, Gain2/1
  Data Type Conversion12/1 -> BytePack1/4
  Data Type Conversion2/1 -> BytePack1/7
  BytePack1/1 -> Subsystem1/1(In1), Mux2/1
  Constant11/1 -> Data Type Conversion2/1
  Constant5/1 -> Data Type Conversion1/1
  Data Type Conversion13/1 -> BytePack1/5
  Constant12/1 -> Data Type Conversion14/1
  Data Type Conversion1/1 -> BytePack1/1
  Constant13/1 -> Data Type Conversion16/1
  Subsystem1/1(Out1) -> Mux2/2
  Gain3/1 -> Data Type Conversion13/1
  Constant10/1 -> Gain3/1

== system AFCToolbox/TEST MOUDLE/TEST POD OUT ==
  Byte Unpack : etargetslib/Byte Unpack  dimensions={1,1,1,1,1,1,1,1,1,1,1,1,1,1,1,1,1,1,1,1}  datatypes={'uint8','uint8','uint8','uint8','uint8','uint8','int16','int16','int16','int16','int16','int16','int16','int16','int16','int16','uint16','uint8','int16','uint8'}  byteAlign=1
      settings: LibrarySourceBlock=embeddedtargetslib/Host Communication/Byte Unpack
  ComXIn1 : $bdroot/DeviceModule/ComXIn  Priority=2  g_sampleTime=0.01  g_comPort=UART7(RS232)  g_baudRate=115200  g_dataSize=32  g_parity=0  g_stopBits=1
  DTComOut : $bdroot/DeviceModule/DTComOut  Priority=8  g_frameType=1  g_outFreq=1  g_comPort=0  g_instName=0  g_id=0
  Data Type Conversion{,1..3} (4 alike) : DataTypeConversion  OutDataTypeStr=double  SaturateOnIntegerOverflow=off  RndMeth=Floor
  Demux : Demux  Outputs=3
  Gain2 : Gain  Gain=0.01
  Mux : Mux  Inputs=3
  Mux3 : Mux  Inputs=3
  Terminator{,1..16} (17 alike) : Terminator
  u16Toi1 : $bdroot/APPModule/u16Toi16
  u16Toi16 : $bdroot/APPModule/u16Toi16
  u16Toi2 : $bdroot/APPModule/u16Toi16
  wires:
  Data Type Conversion/1 -> Gain2/1
  Demux/2 -> Data Type Conversion2/1
  Byte Unpack/18 -> Terminator14/1  "自检结果"
  Byte Unpack/20 -> Terminator16/1  "校验和"
  Mux/1 -> Data Type Conversion/1
  Byte Unpack/17 -> Terminator13/1  "激光测距"
  Byte Unpack/19 -> Terminator15/1  "预留"
  Byte Unpack/5 -> Terminator12/1  "变焦倍数低8位"
  Byte Unpack/6 -> Terminator4/1  "状态反馈信息3"
  Byte Unpack/13 -> Terminator8/1  "预留2"
  Byte Unpack/16 -> Terminator11/1  "方位角速度"
  Data Type Conversion3/1 -> Mux3/3  "方位框架角"
  Byte Unpack/14 -> Terminator9/1  "横滚角速度"
  u16Toi1/1 -> Mux/2
  Gain2/1 -> Demux/1
  Byte Unpack/11 -> u16Toi2/1  "方位框架角"
  Byte Unpack/15 -> Terminator10/1  "俯仰角速度"
  Data Type Conversion1/1 -> Mux3/1  "横滚框架角"
  Data Type Conversion2/1 -> Mux3/2  "俯仰框架角"
  Byte Unpack/4 -> Terminator1/1  "状态信息反馈2"
  Byte Unpack/9 -> u16Toi16/1  "横滚框架角"
  u16Toi16/1 -> Mux/1
  Byte Unpack/8 -> Terminator6/1  "目标脱靶量 Y轴偏移角度"
  Byte Unpack/12 -> Terminator7/1  "预留1"
  Byte Unpack/10 -> u16Toi1/1  "俯仰框架角"
  u16Toi2/1 -> Mux/3
  Demux/3 -> Data Type Conversion3/1
  Byte Unpack/7 -> Terminator5/1  "目标脱靶量 X轴偏移角度"
  Byte Unpack/2 -> Terminator2/1  "同步字2"
  Byte Unpack/3 -> Terminator3/1  "状态信息反馈1"
  ComXIn1/1 -> Byte Unpack/1
  Byte Unpack/1 -> Terminator/1  "同步字1"
  Demux/1 -> Data Type Conversion1/1
  Mux3/1 -> DTComOut/1
